simulink model "Impl_Mower"  (R2026b)
settings: Solver=VariableStepAuto
undefined symbols (not defined in the file or in its folder): P, Ts
libraries: nesl_utility x7, fl_lib x5, ee_lib x4
settings Model: Creator=aomar  LastModifiedBy=aomar

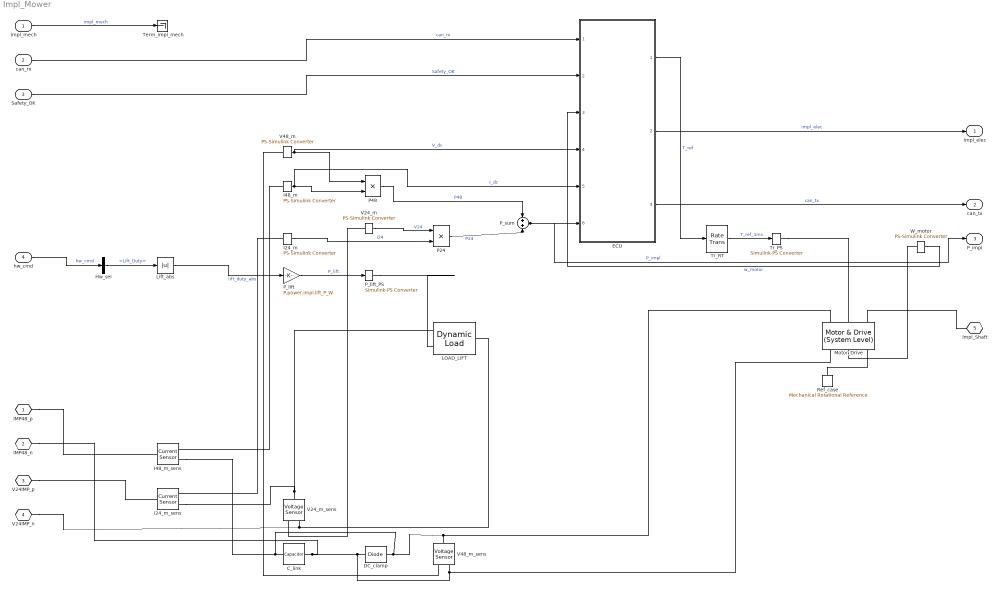
== system Impl_Mower ==
  impl_mech : Inport  OutDataTypeStr=Bus: Bus_ImplMechState  SampleTime=Ts.ctrl
  can_rx : Inport  Port=2  OutDataTypeStr=Bus: Bus_Can1_McuSlow  SampleTime=Ts.can_slow
  Safety_OK : Inport  Port=3  OutDataTypeStr=boolean  SampleTime=Ts.safety
  hw_cmd : Inport  Port=4  OutDataTypeStr=Bus: Bus_PowerHwCmd  SampleTime=Ts.base
  C_link : ee_lib/Passive/Capacitor  cap_option=ee.enum.passive.capacitor.capOption.const  c=P.power.impl.mower.C_link F  Cvec=[1e-05, 1e-06] F  Vvec=[0, 10] V  CV_table_symmetry=ee.enum.passive.capacitor.tableSymmetry.yes  f_vec=[1, 10] kHz  DFext_vec=[.8, 1.2]  enable_C_tol=ee.enum.toleranceApplication.none  averaging_period=0 s  C_tol=5  tol_distribution=ee.enum.toleranceDistribution.uniform  nSigma=4  r=P.power.impl.mower.C_link_esr Ohm  g=0 1/Ohm  enable_operating_limits=ee.enum.enable.no  operating_limit_action=ee.enum.passive.reportOpLim.warn  max_working_voltage_range=[-25, 25] V  power_rating=1 W  maxTemperature=85 degC  thermalEnable=false  thermalMass=1 J/K  i_specify=off  i_priority=None  i=0 A  i_nominal_specify=off  i_nominal_value=1  i_nominal_unit=A  v_specify=off  v_priority=None  v=0 V  v_nominal_specify=off  v_nominal_value=1  v_nominal_unit=V  vc_specify=on  vc_priority=High  vc=0 V  vc_nominal_specify=off  vc_nominal_value=1  vc_nominal_unit=V  T_specify=off  T_priority=None  T=298.15 K  T_nominal_specify=off  T_nominal_value=1  T_nominal_unit=K
  DC_clamp : ee_lib/Semiconductors & Converters/Diode  Vf=0.6 V  Ron=0.3 Ohm  Goff=1e-8 S  N_series=1  N_parallel=1  ZenerEnable=true  BV=P.power.impl.dc_clamp.BV V  Rz=P.power.impl.dc_clamp.Rz Ohm  enable_fault_composite=simscape.enum.onoff.off  i_specify=off  i_priority=None  i=0 A  i_nominal_specify=off  i_nominal_value=1  i_nominal_unit=A  v_specify=off  v_priority=None  v=0 V  v_nominal_specify=off  v_nominal_value=1  v_nominal_unit=V  ModelType=ee.enum.diode.idealModelType.pwl  TableType=ee.enum.diode.tableType.IfMat  IfMat=[.07, .12, .19, 1.75, 4.24, 7.32, 11.2; .16, .3, .72, 2.14, 5.02, 8.35, 13.12] A  VfMat=[.9, 1.15, 1.25, 1.5, 1.75, 2.17, 2.6, 2.85; .58, .68, .75, 1.1, 1.38, 1.77, 2.27, 2.7] V  TjVec=[25, 125] degC  VfVec=[.5, .7, .9, 1.3, 1.7, 2.1, 2.5] V  IfVec=[.1, .2, .5, 1, 2, 4, 7, 10] A  IrMat=[1e-06, 2e-06, 5e-06, 1e-05, 2.5e-05, 5e-05, .0001; 2e-06, 5e-06, 1e-05, 4e-05, 8e-05, .0002, .0005] A  VrMat=[10, 100, 200, 250, 300, 325, 350; 10, 70, 160, 220, 270, 300, 320] V  VrVec=[10, 20, 40, 50, 70, 80, 100] V  IrVec=[1e-06, 2e-06, 5e-06, 1e-05, 2e-05, 5e-05, .0001] A  rec_loss_model=ee.enum.diode.reverseRecoveryModelTabulateUpTo3D.fixed  ErecVal=0 J  scaleWithIandV=true  ErecMat=zeros(2, 3) J  ErecMat3D=zeros(2, 3, 2) J  TjrecVec=[25, 125] degC  IfrecVec=[.1, 1, 10] A  IrecVal=10 A  VrecVal=10 V  VrecVec=[0, 100] V  tFilter=1 / 1000 / 100 s  thermal_network_parameterization=ee.enum.thermalNetworkTopology.junctionCase  Rth=[0, 10] K/W  Rth_Cauer=[1, 3, 10] K/W  Rth_Foster=[.08, .14, .22, .16] K/W  thermal_mass_parameterization=ee.enum.thermalNetwork.timeconstant  thermal_mass=[0, 1] J/K  thermal_mass_Cauer=[.1, .3, 1] J/K  thermal_mass_Foster=[.001, .005, .05, .5] J/K  thermal_time_constant=[0, 10] s  thermal_time_constant_Cauer=[1, 3, 10] s  thermal_time_constant_Foster=[7e-05, .0007, .01, .08] s  thermal_mass_initial_temperatures=[25, 25] degC  thermal_mass_initial_temperatures_Cauer=[25, 25, 25] degC  thermal_mass_initial_temperatures_Foster=[25, 25, 25, 25] degC  junction_thermal_mass=0.01 J/K  junction_temperature_specify=off  junction_temperature_priority=None  junction_temperature=25 degC  junction_temperature_nominal_specify=off  junction_temperature_nominal_value=1  junction_temperature_nominal_unit=degC  ThermalPort=false  ModelTypePhysical=ee.enum.diode.physicalModelType.exponential  prmExp=ee.enum.diode.expParam.useTwo  I12=[.0137, .545] A  V12=[.6, .7] V  IS=1e-12 A  ec=1  I1=0.0137 A  V1=0.6 V  RS=0 Ohm  C_param=ee.enum.diode.capParam.fixed  CJ=0 pF  CJ0=5 pF  Vvec=[.1, 10, 100] V  Cvec=[3.5, 1, .4] pF  VJ=1 V  Mgrad=0.5  FC=0.5  Q_param=ee.enum.diode.recoveryParam.off  iRM=-7.15 A  iF=4 A  didt=-750 A/us  trr_factor=3  trr=115 ns  Qrr=150 nA*s  Vr=-600 V  Ls=150 nH  Erec=0.03 J  TT=50 ns  tau=100 ns  T_param=ee.enum.diode.temperatureParam.off  Tmeas=25 degC  I1_T2=0.245 A  V1_T2=0.5 V  IS_T2=1.25e-7 A  Tmeas2=125 degC  EG_param=ee.enum.diode.egapParam.material_si  EG=1.11 eV  XTI_param=ee.enum.diode.xtiParam.pn  XTI=3  dBVdT=0 V/K  Tdevice=25 degC  i_capacitor_specify=off  i_capacitor_priority=None  i_capacitor=0 A  i_capacitor_nominal_specify=off  i_capacitor_nominal_value=1  i_capacitor_nominal_unit=A  Qj_specify=off  Qj_priority=None  Qj=0 C  Qj_nominal_specify=off  Qj_nominal_value=1  Qj_nominal_unit=uC
  ECU : Subsystem  ReferencedSubsystem=impl_ecu  drv=P.power.impl.mower  impl_type=1
  Hw_sel : BusSelector  OutputSignals=Lift_Duty
  I24_m : nesl_utility/PS-Simulink Converter  PhysicalDomain=network_engine_domain  SubClassName=ps_output  LeftPortType=input  RightPortType=output  PseudoPeriodic=off  Frequencies=[]  VectorFormat=inherit  Unit=A  AffineConversion=off
  I24_m_sens : fl_lib/Electrical/Electrical Sensors/Current Sensor
  I48_m : nesl_utility/PS-Simulink Converter  PhysicalDomain=network_engine_domain  SubClassName=ps_output  LeftPortType=input  RightPortType=output  PseudoPeriodic=off  Frequencies=[]  VectorFormat=inherit  Unit=A  AffineConversion=off
  I48_m_sens : fl_lib/Electrical/Electrical Sensors/Current Sensor
  LOAD_LIFT : ee_lib/Passive/Dynamic Load  load_type=ee.enum.dc_ac.dc  min_supply_voltage=P.power.impl.load_min_V V  pow_min=P.power.lv.load.pow_min W  G_reverse=P.power.lv.load.G_reverse S  deltaV=P.power.lv.load.deltaV V  f0=60 Hz  Vrms_min=200 V  tau=0.01 s  Vrms_ini=300 V  Vang_ini=0 deg
  Lift_abs : Abs  SaturateOnIntegerOverflow=off
  Motor_Drive : ee_lib/Electromechanical/Motor & Drive (System Level)  torque_speed_param=ee.enum.electromech.envelope.tabulated2D  overtorque_param=ee.enum.electromech.overtorque.no  T_t=[.09, .08, .07, 0] N*m  T_t_intermittent=[.36, .32, .28, 0] N*m  T_t_2D=P.power.impl.mower.T_t_2D N*m  T_t_intermittent_2D=[.36, .36, .36; .32, .32, .32; .28, .28, .28; 0, 0, 0] N*m  w_t=P.power.impl.mower.w_t_rpm rpm  vdc_t=P.power.impl.mower.vdc_t V  torque_max=0.1 N*m  power_max=30 W  torque_max_intermittent=0.4 N*m  power_max_intermittent=120 W  time_overtorque=30 s  time_recover=60 s  Tc=P.power.impl.mower.Tc s  EnableSwitch=false  losses_param=ee.enum.electromech.motorAndDrive.lossParameterization.SingleEfficiencyMeasurement  eff=P.power.impl.mower.eff  w_eff=P.power.impl.mower.w_eff_rpm rpm  T_eff=P.power.impl.mower.T_eff N*m  Piron=P.power.impl.mower.Piron W  Pbase=P.power.impl.mower.Pbase W  w_eff_vec=[-8000, -4000, 0, 4000, 8000] rpm  T_eff_vec=[0, .03, .06, .09] N*m  v_eff_vec=[100, 250, 400] V  losses_mat=[1.49, 1.67, 2.21, 3.1; .42, .69, 1.14, 2.03; .06, .24, .78, 1.68; .42, .69, 1.14, 2.03; 1.49, 1.67, 2.21, 3.1] W  efficiency_mat=[95, 95, 95, 95; 95, 95, 95, 95; 95, 95, 95, 95; 95, 95, 95, 95; 95, 95, 95, 95]  losses_mat_3D=ones(5, 4, 3) W  efficiency_mat_3D=95 * ones(5, 4, 3)  Res=0 Ohm  J=P.power.impl.mower.J_motor kg*m^2  lam=P.power.impl.mower.lam N*m*s/rad  speed0=0 rpm  faulted_specify=off  faulted_priority=None  faulted=0  faulted_nominal_specify=off  faulted_nominal_value=1  faulted_nominal_unit=1  isSwitchedOff_specify=off  isSwitchedOff_priority=None  isSwitchedOff=0  isSwitchedOff_nominal_specify=off  isSwitchedOff_nominal_value=1  isSwitchedOff_nominal_unit=1  torqueLimitContinuous_specify=off  torqueLimitContinuous_priority=None  torqueLimitContinuous=0 N*m  torqueLimitContinuous_nominal_specify=off  torqueLimitContinuous_nominal_value=1  torqueLimitContinuous_nominal_unit=N*m  TabulateLossesForMultipleTemperatures=false  alpha=3.93e-3 1/K  Tmeas=25 degC  TmeasVec=[25, 75, 125] degC  Tmeas2=125 degC  losses_mat_T2=[1.49, 1.74, 2.49, 3.74; .42, .67, 1.42, 2.67; .06, .31, 1.06, 2.31; .42, .67, 1.42, 2.67; 1.49, 1.74, 2.49, 3.74] W  efficiency_mat_T2=[95, 95, 95, 95; 95, 95, 95, 95; 95, 95, 95, 95; 95, 95, 95, 95; 95, 95, 95, 95]  losses_mat_3D_T2=ones(5, 4, 3) W  efficiency_mat_3D_T2=95 * ones(5, 4, 3)  lossesMatMultipleTemperatures=ones(5, 4, 3) W  efficiencyMatMultipleTemperatures=95 * ones(5, 4, 3)  lossesMat4DMultipleTemperatures=ones(5, 4, 3, 3) W  efficiencyMat4DMultipleTemperatures=95 * ones(5, 4, 3, 3)  thermal_mass=100 J/K  initial_temperature=25 degC
  P24 : Product
  P48 : Product
  P_lift : Gain  Gain=P.power.impl.lift_P_W
  P_lift_PS : nesl_utility/Simulink-PS Converter  PhysicalDomain=network_engine_domain  SubClassName=ps_input  LeftPortType=input  RightPortType=output  PseudoPeriodic=off  Frequencies=[]  NoiseDistribution=none  NoiseParameters=[]  Unit=W  AffineConversion=off  FilteringAndDerivatives=zero  SimscapeFilterOrder=1  InputFilterTimeConstant=0.001  UdotUserProvided=0
  P_sum : Sum
  Ref_case : fl_lib/Mechanical/Rotational Elements/Mechanical Rotational Reference
  Term_impl_mech : Terminator
  Tr_PS : nesl_utility/Simulink-PS Converter  PhysicalDomain=network_engine_domain  SubClassName=ps_input  LeftPortType=input  RightPortType=output  PseudoPeriodic=off  Frequencies=[]  NoiseDistribution=none  NoiseParameters=[]  Unit=N*m  AffineConversion=off  FilteringAndDerivatives=zero  SimscapeFilterOrder=1  InputFilterTimeConstant=0.001  UdotUserProvided=0
  Tr_RT : RateTransition  OutPortSampleTime=Ts.base
  V24_m : nesl_utility/PS-Simulink Converter  PhysicalDomain=network_engine_domain  SubClassName=ps_output  LeftPortType=input  RightPortType=output  PseudoPeriodic=off  Frequencies=[]  VectorFormat=inherit  Unit=V  AffineConversion=off
  V24_m_sens : fl_lib/Electrical/Electrical Sensors/Voltage Sensor
  V48_m : nesl_utility/PS-Simulink Converter  PhysicalDomain=network_engine_domain  SubClassName=ps_output  LeftPortType=input  RightPortType=output  PseudoPeriodic=off  Frequencies=[]  VectorFormat=inherit  Unit=V  AffineConversion=off
  V48_m_sens : fl_lib/Electrical/Electrical Sensors/Voltage Sensor
  W_motor : nesl_utility/PS-Simulink Converter  PhysicalDomain=network_engine_domain  SubClassName=ps_output  LeftPortType=input  RightPortType=output  PseudoPeriodic=off  Frequencies=[]  VectorFormat=inherit  Unit=rad/s  AffineConversion=off
  IMP48_p : PMIOPort  Side=Left  ConnectionType=Connection: foundation.electrical.electrical
  IMP48_n : PMIOPort  Port=2  Side=Left  ConnectionType=Connection: foundation.electrical.electrical
  V24IMP_p : PMIOPort  Port=3  Side=Left  ConnectionType=Connection: foundation.electrical.electrical
  V24IMP_n : PMIOPort  Port=4  Side=Left  ConnectionType=Connection: foundation.electrical.electrical
  Impl_Shaft : PMIOPort  Port=5  Side=Right  ConnectionType=Connection: foundation.mechanical.rotational.rotational
  impl_elec : Outport  OutDataTypeStr=Bus: Bus_ImplElecState
  can_tx : Outport  Port=2  OutDataTypeStr=Bus: Bus_Can1_Impl
  P_impl : Outport  Port=3  OutDataTypeStr=double
  wires:
  impl_mech/1 -> Term_impl_mech/1  "impl_mech"
  can_rx/1 -> ECU/1  "can_rx"
  Safety_OK/1 -> ECU/2  "Safety_OK"
  hw_cmd/1 -> Hw_sel/1  "hw_cmd"
  Hw_sel/1 -> Lift_abs/1  "<Lift_Duty>"
  Lift_abs/1 -> P_lift/1  "lift_duty_abs"
  V48_m/1 -> P48/1, ECU/4  "V_dc"
  I48_m/1 -> P48/2, ECU/5  "I_dc"
  I24_m/1 -> P24/2  "I24"
  P_lift/1 -> P_lift_PS/1  "P_lift"
  V24_m/1 -> P24/1  "V24"
  P48/1 -> P_sum/1  "P48"
  P24/1 -> P_sum/2  "P24"
  P_sum/1 -> P_impl/1, ECU/6  "P_impl"
  ECU/1 -> Tr_RT/1  "T_ref"
  ECU/2 -> impl_elec/1  "impl_elec"
  ECU/3 -> can_tx/1  "can_tx"
  Tr_RT/1 -> Tr_PS/1  "T_ref_1ms"
  W_motor/1 -> ECU/3  "w_motor"
  connections:
  C_link/LConn1 -- I48_m_sens/RConn2 -- DC_clamp/RConn1 -- V48_m_sens/LConn1 -- Motor_Drive/LConn1
  C_link/RConn1 -- IMP48_n/RConn1 -- DC_clamp/LConn1 -- V48_m_sens/RConn2 -- Motor_Drive/RConn1
  I24_m/LConn1 -- I24_m_sens/RConn1
  V24IMP_p/RConn1 -- I24_m_sens/LConn1
  V24_m_sens/LConn1 -- I24_m_sens/RConn2 -- LOAD_LIFT/LConn1
  I48_m/LConn1 -- I48_m_sens/RConn1
  IMP48_p/RConn1 -- I48_m_sens/LConn1
  Motor_Drive/LConn3 -- Impl_Shaft/RConn1
  P_lift_PS/RConn1 -- LOAD_LIFT/LConn2
  V24_m_sens/RConn2 -- V24IMP_n/RConn1 -- LOAD_LIFT/RConn1
  Tr_PS/RConn1 -- Motor_Drive/LConn2
  W_motor/LConn1 -- Motor_Drive/RConn2
  Ref_case/LConn1 -- Motor_Drive/RConn3
  V24_m/LConn1 -- V24_m_sens/RConn1
  V48_m/LConn1 -- V48_m_sens/RConn1
